simulink model "TV_Sim_Track_Copia"  (R2025b)
settings: Solver=VariableStepAuto  StartTime=0.0  StopTime=20  RelTol=1e-3
values from neighbouring files (symbols this model uses):
  Ki_array = zeros(size(Vx_array))    [PID_analysis.m]    (also in PID_tuning.m)
  psi_ref = theta + pi/2    [init_skidpad.m]
  s_ref = linspace(0, circonferenza, 200)    [init_skidpad.m]
  Vx_array = 1:1:30    [PID_analysis.m]    (also in PID_tuning.m)
  x_ref = R * cos(theta)    [init_skidpad.m]
  y_ref = R * sin(theta)    [init_skidpad.m]
undefined symbols (not defined in the file or in its folder): vp
libraries: slpidlib x3
(part 1 of 2)
settings Model: Creator=roly2  LastModifiedBy=HP

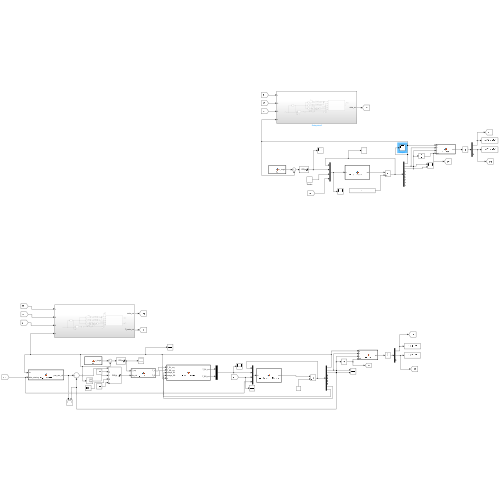
[thumbnail: Simulink's stored preview of the top-level diagram]
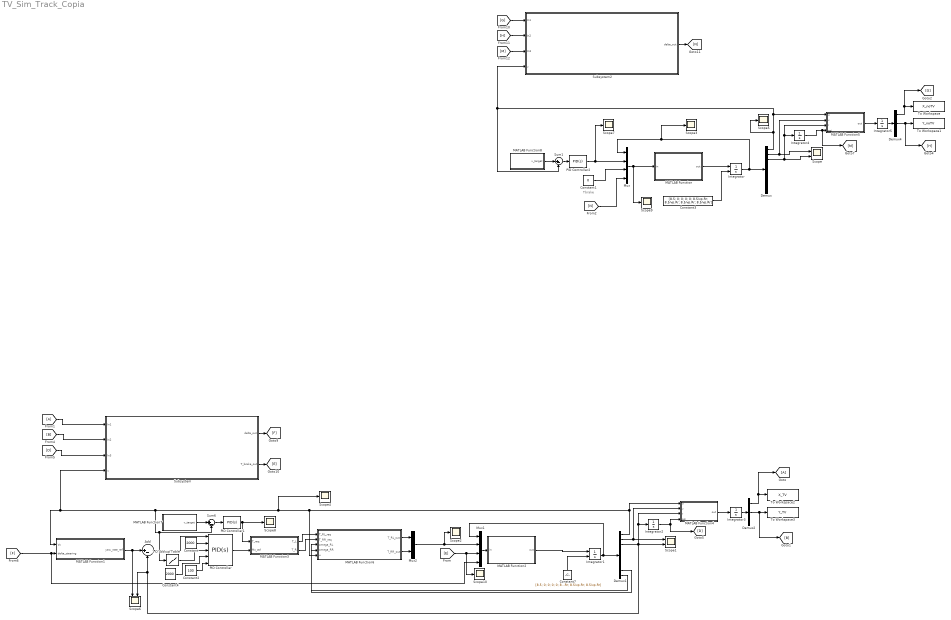
== system TV_Sim_Track_Copia ==
  note: Tbrake
  1-D Lookup Table : Lookup_n-D  NumberOfTableDimensions=1  BreakpointsForDimension1=Vx_array  Table=Ki_array  InternalRulePriority=Speed  RndMeth=Simplest
  Add : Sum  Inputs=|+-
  Constant : Constant  Value=2000
  Constant1 : Constant  Value=0
  Constant2 : Constant  Value=100
  Constant3 : Constant  Value=[8.5; 0; 0; 0; 0; 8.5/vp.Rr; 8.5/vp.Rr; 8.5/vp.Rr; 8.5/vp.Rr]
  Constant4 : Constant  Value=2000
  Constant7 : Constant  Value=[8.5; 0; 0; 0; 0; 8.5/vp.Rr; 8.5/vp.Rr; 8.5/vp.Rr; 8.5/vp.Rr]
  Demux : Demux  Outputs=9
  Demux1 : Demux  Outputs=9
  Demux2 : Demux  Outputs=3
  Demux4 : Demux  Outputs=3
  From1 : From
  Goto : Goto
  Integrator : Integrator  InitialConditionSource=external
  Integrator1 : Integrator  InitialConditionSource=external
  Integrator{2..5} (4 alike) : Integrator
  MATLAB Function : MATLAB Function  TreatAsAtomicUnit=on
  MATLAB Function1 : MATLAB Function  TreatAsAtomicUnit=on
  MATLAB Function2 : MATLAB Function  TreatAsAtomicUnit=on
  MATLAB Function3 : MATLAB Function  TreatAsAtomicUnit=on
  MATLAB Function4 : MATLAB Function  TreatAsAtomicUnit=on
  MATLAB Function5 : MATLAB Function  TreatAsAtomicUnit=on
  MATLAB Function6 : MATLAB Function  TreatAsAtomicUnit=on
  MATLAB Function7 : MATLAB Function  TreatAsAtomicUnit=on
  MATLAB Function8 : MATLAB Function  TreatAsAtomicUnit=on
  Mux : Mux
  Mux1 : Mux
  Mux2 : Mux  Inputs=2
  PID Controller : slpidlib/PID Controller  Controller=PID  Form=Parallel  TimeDomain=Continuous-time  UseExternalTs=off  SampleTime=-1  IntegratorMethod=Forward Euler  FilterMethod=Forward Euler  ControllerParametersSource=external  P=1500  I=12000  UseKiTs=off  D=0  UseExternalDerivativeSource=off  N=100  UseFilter=on  TunerSelectOption=Transfer Function Based (PID Tuner App)  ZeroCross=off  InitialConditionSource=internal  InitialConditionForIntegrator=0  InitialConditionForFilter=0  DifferentiatorICPrevScaledInput=0  ExternalReset=none  TrackingMode=off  Kt=1  LimitOutput=on  SatLimitsSource=internal  UpperSaturationLimit=1000  LowerSaturationLimit=-1000  LinearizeAsGain=on  AntiWindupMode=clamping  Kb=1  LimitIntegrator=off  UpperIntegratorSaturationLimit=inf  LowerIntegratorSaturationLimit=-inf  POutMin=[]  POutMax=[]  IOutMin=[]  IOutMax=[]  DOutMin=[]  DOutMax=[]  NOutMin=[]  NOutMax=[]  SumOutMin=[]  SumOutMax=[]  SaturationOutMin=[]  SaturationOutMax=[]  PParamMin=[]  PParamMax=[]  IParamMin=[]  IParamMax=[]  DParamMin=[]  DParamMax=[]  NParamMin=[]  NParamMax=[]  KbParamMin=[]  KbParamMax=[]  KtParamMin=[]  KtParamMax=[]  KbOutMin=[]  KbOutMax=[]  KtOutMin=[]  KtOutMax=[]  IntegratorOutMin=[]  IntegratorOutMax=[]  FilterOutMin=[]  FilterOutMax=[]  SumI1OutMin=[]  SumI1OutMax=[]  SumI2OutMin=[]  SumI2OutMax=[]  SumI3OutMin=[]  SumI3OutMax=[]  SumI4OutMin=[]  SumI4OutMax=[]  SumDOutMin=[]  SumDOutMax=[]  DifferentiatorOutMin=[]  DifferentiatorOutMax=[]  FilterDiffOutCoefMin=[]  FilterDiffOutCoefMax=[]  ReciprocalOutMin=[]  ReciprocalOutMax=[]  SumDenOutMin=[]  SumDenOutMax=[]  SumNumOutMin=[]  SumNumOutMax=[]  DivideOutMin=[]  DivideOutMax=[]  UdiffTsProdOutMin=[]  UdiffTsProdOutMax=[]  NTsProdOutMin=[]  NTsProdOutMax=[]  UintegralTsProdOutMin=[]  UintegralTsProdOutMax=[]  UngainTsProdOutMin=[]  UngainTsProdOutMax=[]  ClampingZeroOutDataTypeStr=Inherit: Inherit via back propagation  ClampingZeroOutMin=[]  ClampingZeroOutMax=[]  FilterDenConstantOutDataTypeStr=Inherit: Inherit via back propagation  FilterDenConstantOutMin=[]  FilterDenConstantOutMax=[]  PCopyOutDataTypeStr=Inherit: Inherit via back propagation  PCopyOutMin=[]  PCopyOutMax=[]  NCopyOutDataTypeStr=Inherit: Inherit via back propagation  NCopyOutMin=[]  NCopyOutMax=[]  IntegratorContinuousStateAttributes=''  IntegratorStateMustResolveToSignalObject=off  IntegratorRTWStateStorageClass=Auto  FilterContinuousStateAttributes=''  FilterStateMustResolveToSignalObject=off  FilterRTWStateStorageClass=Auto  ParallelPVariant=ExternalParameters  IdealPVariant=Disabled  IVariant=ExternalParameters  DVariant=ExternalParameters  IntegratorVariant=Continuous  SatVariant=Enabled  AWVariant=ContClampingParallel  PCopyVariant=Disabled  TRVariant=Disabled  FdbkBlocksVariant=Forward  IdealPFdbkVariant=Disabled  SatFdbkVariant=Disabled  DerivativeFilterVariant=ContFilter  NVariant=ExternalParameters  NCopyVariant=Disabled  FilterICVariant=InternalICsFilter  IntegratorICVariant=InternalICs  ExternalResetVariant=Disabled  TRSumVariant=Passthrough  SumFdbkVariant=Disabled  SumVariant=Sum_PID  TsampFilterVariant=InternalTs  TsampNgainVariant=Passthrough  TsampIntegralVariant=Disabled_SignalSpec  ExternalSaturationOutDataTypeStr=Inherit: Same as second input  DerivativeSourceVariant=ErrorSignal  PreIntVariant=InternalPreInt
  PID Controller1 : slpidlib/PID Controller  Controller=PID  Form=Parallel  TimeDomain=Continuous-time  UseExternalTs=off  SampleTime=-1  IntegratorMethod=Forward Euler  FilterMethod=Forward Euler  ControllerParametersSource=internal  P=2000  I=3  UseKiTs=off  D=0  UseExternalDerivativeSource=off  N=100  UseFilter=on  TunerSelectOption=Transfer Function Based (PID Tuner App)  InitialConditionSource=internal  InitialConditionForIntegrator=0  InitialConditionForFilter=0  DifferentiatorICPrevScaledInput=0  ExternalReset=none  TrackingMode=off  Kt=1  LimitOutput=on  SatLimitsSource=internal  UpperSaturationLimit=800  LowerSaturationLimit=-8000  LinearizeAsGain=on  AntiWindupMode=clamping  Kb=1  LimitIntegrator=off  UpperIntegratorSaturationLimit=inf  LowerIntegratorSaturationLimit=-inf  POutMin=[]  POutMax=[]  IOutMin=[]  IOutMax=[]  DOutMin=[]  DOutMax=[]  NOutMin=[]  NOutMax=[]  SumOutMin=[]  SumOutMax=[]  SaturationOutMin=[]  SaturationOutMax=[]  PParamMin=[]  PParamMax=[]  IParamMin=[]  IParamMax=[]  DParamMin=[]  DParamMax=[]  NParamMin=[]  NParamMax=[]  KbParamMin=[]  KbParamMax=[]  KtParamMin=[]  KtParamMax=[]  KbOutMin=[]  KbOutMax=[]  KtOutMin=[]  KtOutMax=[]  IntegratorOutMin=[]  IntegratorOutMax=[]  FilterOutMin=[]  FilterOutMax=[]  SumI1OutMin=[]  SumI1OutMax=[]  SumI2OutMin=[]  SumI2OutMax=[]  SumI3OutMin=[]  SumI3OutMax=[]  SumI4OutMin=[]  SumI4OutMax=[]  SumDOutMin=[]  SumDOutMax=[]  DifferentiatorOutMin=[]  DifferentiatorOutMax=[]  FilterDiffOutCoefMin=[]  FilterDiffOutCoefMax=[]  ReciprocalOutMin=[]  ReciprocalOutMax=[]  SumDenOutMin=[]  SumDenOutMax=[]  SumNumOutMin=[]  SumNumOutMax=[]  DivideOutMin=[]  DivideOutMax=[]  UdiffTsProdOutMin=[]  UdiffTsProdOutMax=[]  NTsProdOutMin=[]  NTsProdOutMax=[]  UintegralTsProdOutMin=[]  UintegralTsProdOutMax=[]  UngainTsProdOutMin=[]  UngainTsProdOutMax=[]  ClampingZeroOutDataTypeStr=Inherit: Inherit via back propagation  ClampingZeroOutMin=[]  ClampingZeroOutMax=[]  FilterDenConstantOutDataTypeStr=Inherit: Inherit via back propagation  FilterDenConstantOutMin=[]  FilterDenConstantOutMax=[]  PCopyOutDataTypeStr=Inherit: Inherit via back propagation  PCopyOutMin=[]  PCopyOutMax=[]  NCopyOutDataTypeStr=Inherit: Inherit via back propagation  NCopyOutMin=[]  NCopyOutMax=[]  IntegratorContinuousStateAttributes=''  IntegratorStateMustResolveToSignalObject=off  IntegratorRTWStateStorageClass=Auto  FilterContinuousStateAttributes=''  FilterStateMustResolveToSignalObject=off  FilterRTWStateStorageClass=Auto  ParallelPVariant=InternalParameters  IdealPVariant=Disabled  IVariant=InternalParameters  DVariant=InternalParameters  IntegratorVariant=Continuous  SatVariant=Enabled  AWVariant=ContClampingParallel  PCopyVariant=Disabled  TRVariant=Disabled  FdbkBlocksVariant=Forward  IdealPFdbkVariant=Disabled  SatFdbkVariant=Disabled  DerivativeFilterVariant=ContFilter  NVariant=InternalParameters  NCopyVariant=Disabled  FilterICVariant=InternalICsFilter  IntegratorICVariant=InternalICs  ExternalResetVariant=Disabled  TRSumVariant=Passthrough  SumFdbkVariant=Disabled  SumVariant=Sum_PID  TsampFilterVariant=InternalTs  TsampNgainVariant=Passthrough  TsampIntegralVariant=Disabled_SignalSpec  ExternalSaturationOutDataTypeStr=Inherit: Same as second input  DerivativeSourceVariant=ErrorSignal  PreIntVariant=InternalPreInt
  PID Controller2 : slpidlib/PID Controller  Controller=PID  Form=Parallel  TimeDomain=Continuous-time  UseExternalTs=off  SampleTime=-1  IntegratorMethod=Forward Euler  FilterMethod=Forward Euler  ControllerParametersSource=internal  P=50  I=3  UseKiTs=off  D=0  UseExternalDerivativeSource=off  N=100  UseFilter=on  TunerSelectOption=Transfer Function Based (PID Tuner App)  InitialConditionSource=internal  InitialConditionForIntegrator=0  InitialConditionForFilter=0  DifferentiatorICPrevScaledInput=0  ExternalReset=none  TrackingMode=off  Kt=1  LimitOutput=on  SatLimitsSource=internal  UpperSaturationLimit=800  LowerSaturationLimit=-8000  LinearizeAsGain=on  AntiWindupMode=clamping  Kb=1  LimitIntegrator=off  UpperIntegratorSaturationLimit=inf  LowerIntegratorSaturationLimit=-inf  POutMin=[]  POutMax=[]  IOutMin=[]  IOutMax=[]  DOutMin=[]  DOutMax=[]  NOutMin=[]  NOutMax=[]  SumOutMin=[]  SumOutMax=[]  SaturationOutMin=[]  SaturationOutMax=[]  PParamMin=[]  PParamMax=[]  IParamMin=[]  IParamMax=[]  DParamMin=[]  DParamMax=[]  NParamMin=[]  NParamMax=[]  KbParamMin=[]  KbParamMax=[]  KtParamMin=[]  KtParamMax=[]  KbOutMin=[]  KbOutMax=[]  KtOutMin=[]  KtOutMax=[]  IntegratorOutMin=[]  IntegratorOutMax=[]  FilterOutMin=[]  FilterOutMax=[]  SumI1OutMin=[]  SumI1OutMax=[]  SumI2OutMin=[]  SumI2OutMax=[]  SumI3OutMin=[]  SumI3OutMax=[]  SumI4OutMin=[]  SumI4OutMax=[]  SumDOutMin=[]  SumDOutMax=[]  DifferentiatorOutMin=[]  DifferentiatorOutMax=[]  FilterDiffOutCoefMin=[]  FilterDiffOutCoefMax=[]  ReciprocalOutMin=[]  ReciprocalOutMax=[]  SumDenOutMin=[]  SumDenOutMax=[]  SumNumOutMin=[]  SumNumOutMax=[]  DivideOutMin=[]  DivideOutMax=[]  UdiffTsProdOutMin=[]  UdiffTsProdOutMax=[]  NTsProdOutMin=[]  NTsProdOutMax=[]  UintegralTsProdOutMin=[]  UintegralTsProdOutMax=[]  UngainTsProdOutMin=[]  UngainTsProdOutMax=[]  ClampingZeroOutDataTypeStr=Inherit: Inherit via back propagation  ClampingZeroOutMin=[]  ClampingZeroOutMax=[]  FilterDenConstantOutDataTypeStr=Inherit: Inherit via back propagation  FilterDenConstantOutMin=[]  FilterDenConstantOutMax=[]  PCopyOutDataTypeStr=Inherit: Inherit via back propagation  PCopyOutMin=[]  PCopyOutMax=[]  NCopyOutDataTypeStr=Inherit: Inherit via back propagation  NCopyOutMin=[]  NCopyOutMax=[]  IntegratorContinuousStateAttributes=''  IntegratorStateMustResolveToSignalObject=off  IntegratorRTWStateStorageClass=Auto  FilterContinuousStateAttributes=''  FilterStateMustResolveToSignalObject=off  FilterRTWStateStorageClass=Auto  ParallelPVariant=InternalParameters  IdealPVariant=Disabled  IVariant=InternalParameters  DVariant=InternalParameters  IntegratorVariant=Continuous  SatVariant=Enabled  AWVariant=ContClampingParallel  PCopyVariant=Disabled  TRVariant=Disabled  FdbkBlocksVariant=Forward  IdealPFdbkVariant=Disabled  SatFdbkVariant=Disabled  DerivativeFilterVariant=ContFilter  NVariant=InternalParameters  NCopyVariant=Disabled  FilterICVariant=InternalICsFilter  IntegratorICVariant=InternalICs  ExternalResetVariant=Disabled  TRSumVariant=Passthrough  SumFdbkVariant=Disabled  SumVariant=Sum_PID  TsampFilterVariant=InternalTs  TsampNgainVariant=Passthrough  TsampIntegralVariant=Disabled_SignalSpec  ExternalSaturationOutDataTypeStr=Inherit: Same as second input  DerivativeSourceVariant=ErrorSignal  PreIntVariant=InternalPreInt
  Scope : Scope  NumInputPorts=2
      settings: ActiveDisplayYMinimum=-0.036171963019396312  ActiveDisplayYMaximum=0.32541321822804137
  Scope1 : Scope  NumInputPorts=2
      settings: ActiveDisplayYMinimum=-0.20199456045323017  ActiveDisplayYMaximum=0.60254469008079159
  Scope{2..5,7..10} (8 alike) : Scope
      Scope10 settings: ActiveDisplayYMinimum=-1  ActiveDisplayYMaximum=1  DataLoggingVariableName=ScopeData10
      Scope2 settings: ActiveDisplayYMinimum=-54.565881529047566  ActiveDisplayYMaximum=241.09293376142816  DataLoggingVariableName=ScopeData2
      Scope3 settings: ActiveDisplayYMinimum=-12.645443098724071  ActiveDisplayYMaximum=111.73678774278743  DataLoggingVariableName=ScopeData3
      Scope4 settings: ActiveDisplayYMinimum=-115.18294853972765  ActiveDisplayYMaximum=23.840986492179059  DataLoggingVariableName=ScopeData4
      Scope5 settings: ActiveDisplayYMinimum=7.8538069739436995  ActiveDisplayYMaximum=8.5717992251173669  DataLoggingVariableName=ScopeData5
      Scope7 settings: ActiveDisplayYMinimum=-3.3845352985098125  ActiveDisplayYMaximum=43.431126970490176  DataLoggingVariableName=ScopeData7
      Scope8 settings: ActiveDisplayYMinimum=-132.10801998182529  ActiveDisplayYMaximum=486.27732365321947  DataLoggingVariableName=ScopeData8
      Scope9 settings: ActiveDisplayYMinimum=-8.521232283481865  ActiveDisplayYMaximum=11.017708574192625  DataLoggingVariableName=ScopeData9
  Scope6 : Scope  NumInputPorts=2
      settings: ActiveDisplayYMinimum=-0.14426470588235293  ActiveDisplayYMaximum=1.2983823529411767  DataLoggingVariableName=ScopeData6
  Subsystem : Subsystem
  Subsystem2 : Subsystem
  Sum1 : Sum  Inputs=|+-
  Sum6 : Sum  Inputs=|+-
  To Workspace : ToWorkspace  VariableName=X_noTV  SaveFormat=Timeseries  SampleTime=-1
      settings: Save2DSignal=2-D array (concatenate along first dimension)
  To Workspace1 : ToWorkspace  VariableName=Y_noTV  SaveFormat=Timeseries  SampleTime=-1
      settings: Save2DSignal=2-D array (concatenate along first dimension)
  To Workspace2 : ToWorkspace  VariableName=X_TV  SaveFormat=Timeseries  SampleTime=-1
      settings: Save2DSignal=2-D array (concatenate along first dimension)
  To Workspace3 : ToWorkspace  VariableName=Y_TV  SaveFormat=Timeseries  SampleTime=-1
      settings: Save2DSignal=2-D array (concatenate along first dimension)
  wires:
  Add/1 -> PID Controller/1
  Constant7/1 -> Integrator1/2
  Demux2/1 -> Goto/1, To Workspace2/1
  MATLAB Function2/1(out) -> Integrator1/1
  Integrator3/1 -> Demux2/1
  Integrator1/1 -> Demux1/1, Mux1/1
  Demux2/2 -> [B], To Workspace3/1
  Integrator2/1 -> [D], MATLAB Function4/4(psi)
  Demux1/2 -> MATLAB Function4/2(v), Scope1/1
  MATLAB Function4/1(out) -> Integrator3/1
  Mux1/1 -> MATLAB Function2/1(in)
  Demux1/3 -> Add/2, Scope6/2, Integrator2/1, MATLAB Function4/3(r), Scope1/2
  Integrator4/1 -> [M], MATLAB Function5/4(psi)
  Integrator5/1 -> Demux4/1
  Integrator/1 -> Demux/1, Scope3/1, Mux/1
  Constant1/1 -> Mux/3
  MATLAB Function5/1(out) -> Integrator5/1
  Demux4/2 -> [H], To Workspace1/1
  Mux/1 -> Scope9/1, MATLAB Function/1(in)
  Constant3/1 -> Integrator/2
  MATLAB Function/1(out) -> Integrator/1
  Demux/3 -> Integrator4/1, MATLAB Function5/3(r), Scope/2
  Demux4/1 -> [G], To Workspace/1
  Demux/2 -> MATLAB Function5/2(v), Scope/1
  PID Controller/1 -> MATLAB Function3/2(Mz_ctrl)
  Mux2/1 -> Mux1/2, Scope2/1
  MATLAB Function3/2(T_R) -> MATLAB Function6/2(T_RR_req)
  MATLAB Function3/1(T_L) -> MATLAB Function6/1(T_RL_req)
  Demux1/8 -> MATLAB Function6/3(omega_RL)
  Demux1/9 -> MATLAB Function6/4(omega_RR)
  MATLAB Function6/1(T_RL_out) -> Mux2/1
  MATLAB Function6/2(T_RR_out) -> Mux2/2
  MATLAB Function1/1(yaw_rate_ref) -> Add/1, Scope6/1
  [F] -> Mux1/4, MATLAB Function1/2(delta_steering)
  MATLAB Function7/1(v_target) -> Sum6/1
  Sum6/1 -> PID Controller1/1
  PID Controller1/1 -> Scope8/1, MATLAB Function3/1(T_req)
  [N] -> Mux/4
  PID Controller2/1 -> Mux/2, Scope7/1
  Sum1/1 -> PID Controller2/1
  MATLAB Function8/1(v_target) -> Sum1/1
  Constant/1 -> PID Controller/2
  1-D Lookup Table/1 -> PID Controller/3
  Constant2/1 -> PID Controller/5
  Demux1/1 -> MATLAB Function4/1(u), 1-D Lookup Table/1, Sum6/2, MATLAB Function1/1(Vx), Subsystem/4(v), Scope4/1, MATLAB Function6/5(u)
  From1/1 -> Subsystem/1(In1)
  [B] -> Subsystem/2(In2)
  [D] -> Subsystem/3(In3)
  Subsystem/1(delta_out) -> [F]
  Subsystem/2(T_brake_out) -> [E]
  [E] -> Scope10/1, Mux1/3
  [M] -> Subsystem2/3(In3)
  Demux/1 -> Scope5/1, Subsystem2/4(v), Sum1/2, MATLAB Function5/1(u)
  [H] -> Subsystem2/2(In2)
  Subsystem2/1(delta_out) -> [N]
  [G] -> Subsystem2/1(In1)
  Constant4/1 -> PID Controller/4

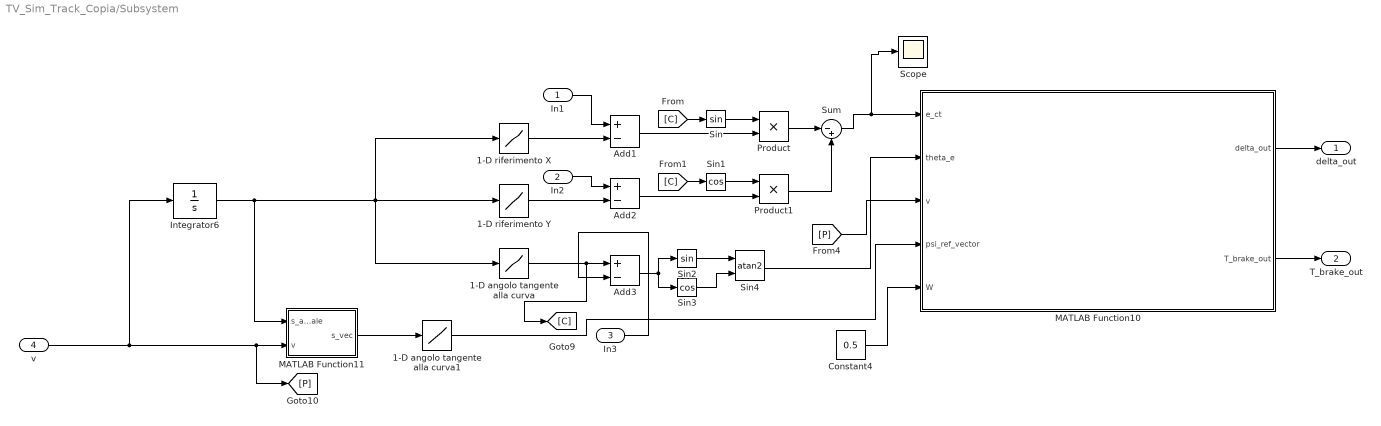
== system TV_Sim_Track_Copia/Subsystem ==
  In1 : Inport
  In2 : Inport  Port=2
  In3 : Inport  Port=3
  v : Inport  Port=4
  1-D angolo tangente alla curva : Lookup_n-D  NumberOfTableDimensions=1  BreakpointsForDimension1=s_ref  Table=psi_ref  ExtrapMethod=Clip  InternalRulePriority=Speed  RndMeth=Simplest
  1-D angolo tangente alla curva1 : Lookup_n-D  NumberOfTableDimensions=1  BreakpointsForDimension1=s_ref  Table=psi_ref  ExtrapMethod=Clip  InternalRulePriority=Speed  RndMeth=Simplest
  1-D riferimento X : Lookup_n-D  NumberOfTableDimensions=1  BreakpointsForDimension1=s_ref  Table=x_ref  ExtrapMethod=Clip  InternalRulePriority=Speed  RndMeth=Simplest
  1-D riferimento Y : Lookup_n-D  NumberOfTableDimensions=1  BreakpointsForDimension1=s_ref  Table=y_ref  ExtrapMethod=Clip  InternalRulePriority=Speed  RndMeth=Simplest
  Add1 : Sum  Inputs=+-
  Add2 : Sum  Inputs=+-
  Add3 : Sum  Inputs=+-
  Constant4 : Constant  Value=0.5
  Integrator6 : Integrator  UpperSaturationLimit=94.2478  LowerSaturationLimit=0
  MATLAB Function10 : MATLAB Function  TreatAsAtomicUnit=on
  MATLAB Function11 : MATLAB Function  TreatAsAtomicUnit=on
  Product : Product
  Product1 : Product
  Scope : Scope
      settings: ActiveDisplayYMinimum=-1  ActiveDisplayYMaximum=1  DataLoggingVariableName=ScopeData11
  Sin : Trigonometry
  Sin1 : Trigonometry  Operator=cos
  Sin2 : Trigonometry
  Sin3 : Trigonometry  Operator=cos
  Sin4 : Trigonometry  Operator=atan2
  Sum : Sum  Inputs=|-+
  delta_out : Outport
  T_brake_out : Outport  Port=2
  wires:
  v/1 -> Integrator6/1, [P], MATLAB Function11/2(v)
  Sin3/1 -> Sin4/2
  In1/1 -> Add1/1
  Sin4/1 -> MATLAB Function10/2(theta_e)
  MATLAB Function10/2(T_brake_out) -> T_brake_out/1
  1-D angolo tangente alla curva/1 -> [C], Add3/1
  [P] -> MATLAB Function10/3(v)
  1-D riferimento Y/1 -> Add2/2
  Sin2/1 -> Sin4/1
  Product/1 -> Sum/1
  [C] -> Sin1/1
  Add2/1 -> Product1/2
  Product1/1 -> Sum/2
  In2/1 -> Add2/1
  1-D angolo tangente alla curva1/1 -> MATLAB Function10/4(psi_ref_vector)
  Sin/1 -> Product/1
  Add3/1 -> Sin3/1, Sin2/1
  Add1/1 -> Product/2
  Sin1/1 -> Product1/1
  MATLAB Function11/1(s_vec) -> 1-D angolo tangente alla curva1/1
  1-D riferimento X/1 -> Add1/2
  In3/1 -> Add3/2
  Sum/1 -> Scope/1, MATLAB Function10/1(e_ct)
  [C] -> Sin/1
  Constant4/1 -> MATLAB Function10/5(W)
  MATLAB Function10/1(delta_out) -> delta_out/1
  Integrator6/1 -> MATLAB Function11/1(s_attuale), 1-D angolo tangente alla curva/1, 1-D riferimento X/1, 1-D riferimento Y/1

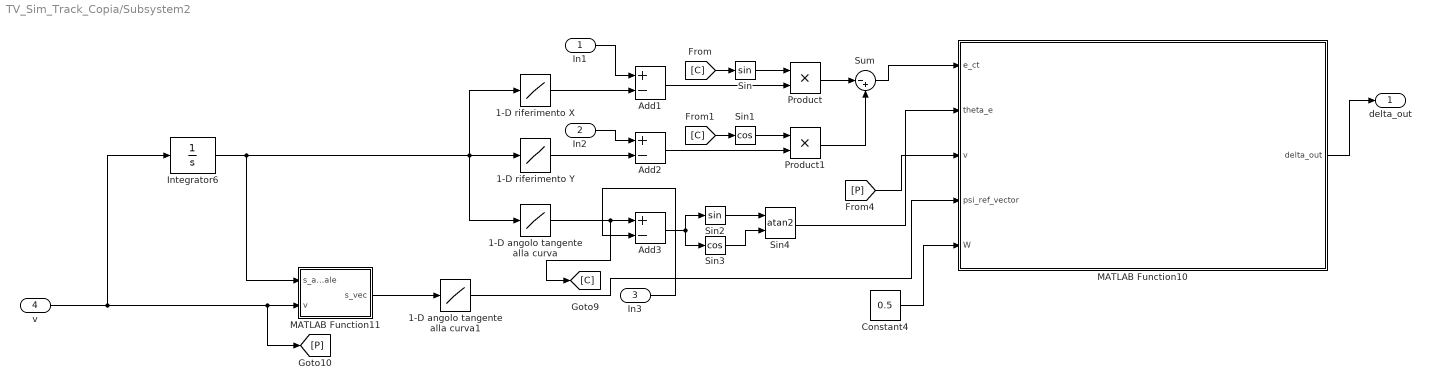
== system TV_Sim_Track_Copia/Subsystem2 ==
  In1 : Inport
  In2 : Inport  Port=2
  In3 : Inport  Port=3
  v : Inport  Port=4
  1-D angolo tangente alla curva : Lookup_n-D  NumberOfTableDimensions=1  BreakpointsForDimension1=s_ref  Table=psi_ref  ExtrapMethod=Clip  InternalRulePriority=Speed  RndMeth=Simplest
  1-D angolo tangente alla curva1 : Lookup_n-D  NumberOfTableDimensions=1  BreakpointsForDimension1=s_ref  Table=psi_ref  ExtrapMethod=Clip  InternalRulePriority=Speed  RndMeth=Simplest
  1-D riferimento X : Lookup_n-D  NumberOfTableDimensions=1  BreakpointsForDimension1=s_ref  Table=x_ref  ExtrapMethod=Clip  InternalRulePriority=Speed  RndMeth=Simplest
  1-D riferimento Y : Lookup_n-D  NumberOfTableDimensions=1  BreakpointsForDimension1=s_ref  Table=y_ref  ExtrapMethod=Clip  InternalRulePriority=Speed  RndMeth=Simplest
  Add1 : Sum  Inputs=+-
  Add2 : Sum  Inputs=+-
  Add3 : Sum  Inputs=+-
  Constant4 : Constant  Value=0.5
  Integrator6 : Integrator  UpperSaturationLimit=94.2478  LowerSaturationLimit=0
  MATLAB Function10 : MATLAB Function  TreatAsAtomicUnit=on
  MATLAB Function11 : MATLAB Function  TreatAsAtomicUnit=on
  Product : Product
  Product1 : Product
  Sin : Trigonometry
  Sin1 : Trigonometry  Operator=cos
  Sin2 : Trigonometry
  Sin3 : Trigonometry  Operator=cos
  Sin4 : Trigonometry  Operator=atan2
  Sum : Sum  Inputs=|-+
  delta_out : Outport
  wires:
  v/1 -> Integrator6/1, [P], MATLAB Function11/2(v)
  Sin3/1 -> Sin4/2
  In1/1 -> Add1/1
  Sin4/1 -> MATLAB Function10/2(theta_e)
  1-D angolo tangente alla curva/1 -> [C], Add3/1
  [P] -> MATLAB Function10/3(v)
  1-D riferimento Y/1 -> Add2/2
  Integrator6/1 -> 1-D angolo tangente alla curva/1, 1-D riferimento X/1, 1-D riferimento Y/1, MATLAB Function11/1(s_attuale)
  Sin2/1 -> Sin4/1
  Product/1 -> Sum/1
  [C] -> Sin1/1
  Add2/1 -> Product1/2
  Product1/1 -> Sum/2
  In2/1 -> Add2/1
  1-D angolo tangente alla curva1/1 -> MATLAB Function10/4(psi_ref_vector)
  Sin/1 -> Product/1
  Add3/1 -> Sin3/1, Sin2/1
  Add1/1 -> Product/2
  Sin1/1 -> Product1/1
  MATLAB Function11/1(s_vec) -> 1-D angolo tangente alla curva1/1
  1-D riferimento X/1 -> Add1/2
  In3/1 -> Add3/2
  Sum/1 -> MATLAB Function10/1(e_ct)
  [C] -> Sin/1
  Constant4/1 -> MATLAB Function10/5(W)
  MATLAB Function10/1(delta_out) -> delta_out/1

== matlab function TV_Sim_Track_Copia/Subsystem/MATLAB Function10 ==
  data: e_ct input; delta_out output; T_brake_out output; theta_e input; v input; psi_ref_vector input; W input
function [delta_out, T_brake_out] = fcn(e_ct, theta_e, v, psi_ref_vector, W)
    % --- PARAMETRI DI CONFIGURAZIONE ---
    N = length(psi_ref_vector); % Numero di punti futuri (es. 10)
    dt = 0.1;                   % Passo temporale della previsione [s]
    
    % Margine di sicurezza: l'auto cercherà di stare entro questo limite
    % Se W=10m, Lat_Limit sarà 4.7m (lasciando 30cm dal bordo)
    Lat_Limit = (W/2) - 0.3; 

    % --- 1. PREVISIONE DEL FUTURO (ORIZZONTE N) ---
    % Inizializziamo le variabili per la simulazione interna
    future_e_ct = zeros(1, N);
    temp_e = e_ct;
    temp_theta = theta_e;
    
for k = 1:N
    % Calcola la differenza angolare
    diff_angle = temp_theta - psi_ref_vector(k);
    
    % CORREZIONE WRAP-AROUND: mantiene l'angolo tra -pi e pi
    diff_angle = atan2(sin(diff_angle), cos(diff_angle));
    
    % Usa l'angolo corretto per la previsione
    temp_e = temp_e + v * sin(diff_angle) * dt;
    future_e_ct(k) = temp_e;
end

    % --- 2. LOGICA DI CONTROLLO STERZO (FEEDBACK) ---
    % Usiamo una base simile allo Stanley per l'inseguimento normale
    k_stanley = 0.5;
    k_soft = 1.0;
    delta_feedback = theta_e - atan2(k_stanley * e_ct, v + k_soft);

    % --- 3. LOGICA DI VINCOLO (THE "HARD" CONSTRAINT) ---
    % Troviamo l'errore massimo previsto nell'orizzonte
    max_predicted_error = max(abs(future_e_ct));
    
    if max_predicted_error > Lat_Limit
        % --- SE L'AUTO PREVEDE DI USCIRE ---
        
        % A. Calcoliamo quanto stiamo violando il limite
        violazione = max_predicted_error - Lat_Limit;
        
        % B. FRENO OBBLIGATORIO: Più la violazione è grande, più frena.
        % Questo riduce v e "stringe" la traiettoria fisicamente.
        T_brake_out = 0; %2500 * violazione; 
        
        % C. STERZO DI EMERGENZA: Aumentiamo il guadagno per chiudere la curva
        delta_out = delta_feedback * (1 + 2 * violazione);
    else
        % --- TRAIETTORIA SICURA ---
        T_brake_out = 0;
        delta_out = delta_feedback;
    end

    % --- 4. SATURAZIONI FISICHE ---
    % Limite sterzo (es. 35 gradi)
    delta_out = max(min(delta_out, 0.6), -0.6);
    
    % Limite frenata massima (Nm)
    T_brake_out = max(min(T_brake_out, 4000), 0);
end

== matlab function TV_Sim_Track_Copia/Subsystem/MATLAB Function11 ==
  data: s_attuale input; s_vec output; v input
function s_vec = fcn(s_attuale, v)
    dt = 0.1; % Passo temporale (prevediamo i prossimi 10 decimi di secondo)
    % Creiamo un vettore: [s, s+v*0.1, s+v*0.2, ..., s+v*0.9]
    s_vec = s_attuale + v * dt * (0:9); 
end

== matlab function TV_Sim_Track_Copia/Subsystem2/MATLAB Function11 ==
  data: s_attuale input; s_vec output; v input
function s_vec = fcn(s_attuale, v)
    dt = 0.1; % Passo temporale (prevediamo i prossimi 10 decimi di secondo)
    % Creiamo un vettore: [s, s+v*0.1, s+v*0.2, ..., s+v*0.9]
    s_vec = s_attuale + v * dt * (0:9); 
end

== matlab function TV_Sim_Track_Copia/MATLAB Function1 ==
  data: Vx input; delta_steering input; yaw_rate_ref output; vp parameter
function yaw_rate_ref = ref_generator(Vx, delta_steering, vp)

% --- 1. PARAMETRI E CONVERSIONI ---
% Stima del coefficiente d'attrito (es. 1.0 asciutto, 0.7 umido)
% In futuro questo valore potrà arrivare da uno stimatore
mu = 1.0;

K_tf_deg = 1150;
K_tr_deg = 1010;
K_tf = K_tf_deg * (180/pi); 
K_tr = K_tr_deg * (180/pi); 

K_us = (vp.m / vp.l)*(vp.a2/K_tf - vp.a1/K_tr);

delta = delta_steering * vp.tau1;

% --- 2. RIFERIMENTO LINEARE (Desired Handling) ---
% Eq. (1) del paper: Comportamento ideale se avessimo grip infinito [cite: 2044]
% Protezione per Vx molto bassi per evitare divisioni per zero instabili
Vx_safe = max(abs(Vx), 1.0);

r_linear = Vx / (vp.l*(1 + K_us * Vx^2)) * delta;

% --- 3. SATURAZIONE FISICA (Safety/Grip Limit) ---
% Il paper spiega che il limite è dato dall'attrito disponibile 
% Massima accelerazione laterale sostenibile (in m/s^2)
ay_max = mu * vp.g;

% Massima velocità di imbardata possibile a questa velocità
% Dalla relazione: ay = V * r  -->  r_max = ay_max / V
r_max_phys = ay_max / Vx_safe;

% --- 4. OUTPUT FINALE (Logica Min/Max) ---
% Il riferimento è il minimo tra quello che "vorrebbe" il pilota (lineare)
% e quello che la fisica "permette" (limite saturato).

% Manteniamo il segno originale della richiesta
sign_r = sign(r_linear);

% Se la richiesta lineare supera il limite fisico, tagliamo al limite.
if abs(r_linear) > r_max_phys
    yaw_rate_ref = sign_r * r_max_phys;
else
    yaw_rate_ref = r_linear;
end

% (Opzionale Avanzato): Per mimare l'esponenziale del paper,
% si potrebbe usare una tanh() per una transizione più morbida vicino al limite,
% ma la saturazione secca (if/else) sopra è più sicura per iniziare.


end

== matlab function TV_Sim_Track_Copia/MATLAB Function ==
  data: in input size=12; out output; vp parameter
function out  = Vehicle_model_NL(in, vp)
% Modello del veicolo non lineare

u = in(1);
v = in(2);
r = in(3);
nu = in(4);
epsilon = in(5);
omega11 = in(6);
omega12 = in(7);
omega21 = in(8);
omega22 = in(9);
% Coppia motrice [Nm]
Tdrive = in(10);
% Coppia frenante [Nm]
Tbrake = in(11);
% Angolo di sterzo [rad]
deltav = in(12);


% ModelloVeicolo_2025/2026

% 2) Definizione dei limiti sugli stati

u_lim = 1/u*[0 vp.Vmax]; % Questo è abbastanza chiaro, in caso va solo cambiata la scalatura
v_lim = 1/v*[-10 10]; % Questo si cerca di tenerlo attorno a 1
r_lim = 1/r*[-10 10]; % Qui mettiamoci un pi/2 
nu_lim = 1/nu*[-0.875 0.875]; %Per skid
%nu_lim = 1/nu*[-1 1]; % Questo in teoria permette di specificare la largezza del circuito, assunta costante. Dovrebbe esserci il modo di mettere una distanza variabile ma è follia, messo a 1
epsilon_lim = 1/epsilon*[-pi/4 pi/4]; % Un po' strano ma in realtà è solo pi/4
% Le velocità angolari abbastanza semplici, fermo al minimo, Vmax/u al massimo
omega11_lim = 1/omega11*[0 vp.Vmax/vp.Rr];
omega12_lim = 1/omega12*[0 vp.Vmax/vp.Rr];
omega21_lim = 1/omega21*[0 vp.Vmax/vp.Rr];
omega22_lim = 1/omega22*[0 vp.Vmax/vp.Rr];

% 3) Raggruppamento

% Vettore degli stati 
X = [u; v; r; nu; epsilon; omega11; omega12; omega21; omega22];
% Limiti
X_lim = [u_lim;v_lim;r_lim;nu_lim;epsilon_lim;omega11_lim;omega12_lim;omega21_lim;omega22_lim];
X_min = X_lim(:,1);
X_max = X_lim(:,2);

% Differernziale similmeccanico aperto ***********
TdriveR = (Tdrive)/2; 
TdriveL = (Tdrive)/2;

% 2) Definizione dei limiti sui controlli + Frenata rigenerativa

TdriveR_lim = 1/TdriveR*[-vp.Tregenmax vp.Tdrivemax];
TdriveL_lim = 1/TdriveL*[-vp.Tregenmax vp.Tdrivemax];
Tbrake_lim = 1/Tbrake*[-vp.Tbrakemax 0];
deltav_lim = 1/deltav*[-pi/2 pi/2];

% 3) Raggruppamento

% Vettore dei controlli
U = [Tdrive; Tbrake; deltav];
% Limiti
U_lim = [TdriveR_lim;TdriveL_lim;Tbrake_lim;deltav_lim];
U_min = U_lim(:,1);
U_max = U_lim(:,2);

% Vincolo ulteriore sulla derivata dei controlli, sfrutta quello definito prima
%duk_ub = duk_ub./U;
%duk_lb = duk_lb./U;
%per ora sono come testo perchè non so quanto valgono queste derivate

% VARIABILI AUSILIARIE

% 1) Definizione simbolica deille variabili ausiliarie

% Trasferimento di carico longitudinale [N]
deltaZ = vp.m*vp.g*vp.h/vp.l;

% Trasferimento di carico laterale anteriore [N]
deltaZ1 = (((vp.kphi1/vp.kphi)*(vp.m*vp.g)*(vp.h-vp.qb)+(vp.m*vp.g*vp.a2/vp.l)*vp.q1+(vp.kphi1*vp.kphi2/vp.kphi)*((vp.m*vp.g*vp.a1/vp.l)*vp.q2/vp.kphi2p-(vp.m*vp.g*vp.a2/vp.l)*vp.q1/vp.kphi1p))*(1/vp.t1));

% Trasferimento di carico laterale posteriore [N]
deltaZ2 = (((vp.kphi1/vp.kphi)*(vp.m*vp.g)*(vp.h-vp.qb)+(vp.m*vp.g*vp.a1/vp.l)*vp.q1+(vp.kphi1*vp.kphi2/vp.kphi)*((vp.m*vp.g*vp.a2/vp.l)*vp.q2/vp.kphi2p-(vp.m*vp.g*vp.a1/vp.l)*vp.q1/vp.kphi1p))*(1/vp.t1));

% 2) Definizione dei limiti sulle variabili ausiliarie

deltaZ_lim = 1/deltaZ*[-2*vp.m*vp.g 2*vp.m*vp.g];
deltaZ1_lim = 1/deltaZ1*[-2*vp.m*vp.g 2*vp.m*vp.g];
deltaZ2_lim = 1/deltaZ2*[-2*vp.m*vp.g 2*vp.m*vp.g];

% 3) Raggruppamento

% Vettore delle variabili ausiliarie 
Zaus = [deltaZ;deltaZ1;deltaZ2];
% Limiti
Zaus_lim = [deltaZ_lim;deltaZ1_lim;deltaZ2_lim];
Zaus_min = Zaus_lim(:,1);
Zaus_max = Zaus_lim(:,2);

% EQUAZIONI 

% 1) Legge di sterzo

delta11 = -vp.delta10+vp.tau1*deltav+vp.eps1*(vp.t1/(2*vp.l))*(vp.t1*deltav)^2;
delta12 = vp.delta10+vp.tau1*deltav-vp.eps1*(vp.t1/(2*vp.l))*(vp.t1*deltav)^2;
delta21 = -vp.delta20+vp.tau2*deltav+vp.eps2*(vp.t2/(2*vp.l))*(vp.t2*deltav)^2;
delta22 = vp.delta20+vp.tau2*deltav-vp.eps2*(vp.t2/(2*vp.l))*(vp.t2*deltav)^2;

% 2) Velocità pneumatici sistema "Body

% FRONT LEFT
Vb11x = u-(r*vp.t1)/2; Vb11y = v+r*vp.a1;
% FRONT RIGHT
Vb12x = u+(r*vp.t1)/2; Vb12y = v+r*vp.a1;
% REAR LEFT
Vb21x = u-(r*vp.t2)/2; Vb21y = v-r*vp.a2;
% REAR RIGHT
Vb22x = u+(r*vp.t2)/2; Vb22y = v-r*vp.a2;

% 3) Angoli di assetto

% FRONT LEFT
beta11 = (v+r*vp.a1)/(u-r*vp.t1/2);
% FRONT RIGHT
beta12 = (v+r*vp.a1)/(u+r*vp.t1/2);
% REAR LEFT
beta21 = (v-r*vp.a2)/(u-r*vp.t2/2);
% REAR RIGHT
beta22 = (v-r*vp.a2)/(u+r*vp.t2/2);

% 3b) Velocità sistema "Wheel"

% FRONT LEFT
Vw11x = [cos(delta11) sin(delta11)]*[Vb11x;Vb11y];
Vw11y = [-sin(delta11) cos(delta11)]*[Vb11x;Vb11y];
% FRONT RIGHT
Vw12x = [cos(delta12) sin(delta12)]*[Vb12x;Vb12y];
Vw12y = [-sin(delta12) cos(delta12)]*[Vb12x;Vb12y];
% REAR LEFT
Vw21x = [cos(delta21) sin(delta21)]*[Vb21x;Vb21y];
Vw21y = [-sin(delta21) cos(delta21)]*[Vb21x;Vb21y];
% REAR RIGHT
Vw22x = [cos(delta22) sin(delta22)]*[Vb22x;Vb22y];
Vw22y = [-sin(delta22) cos(delta22)]*[Vb22x;Vb22y];

% 4) Angoli di deriva

% FRONT LEFT
alpha11 = delta11-beta11;
% FRONT RIGHT
alpha12 = delta12-beta12;
% REAR LEFT
alpha21 = delta21-beta21;
% REAR RIGHT
alpha22 = delta22-beta22;

% 5) Scorrimenti teorici

% Longitudinali
sigmax11 = (((u-r*vp.t1/2)*cos(delta11)+(v+r*vp.a1)*sin(delta11))-omega11*vp.Rr)/(omega11*vp.Rr);
sigmax12 = (((u+r*vp.t1/2)*cos(delta12)+(v+r*vp.a1)*sin(delta12))-omega12*vp.Rr)/(omega12*vp.Rr);
sigmax21 = (((u-r*vp.t2/2)*cos(delta21)+(v-r*vp.a2)*sin(delta21))-omega21*vp.Rr)/(omega21*vp.Rr);
sigmax22 = (((u+r*vp.t2/2)*cos(delta22)+(v-r*vp.a2)*sin(delta22))-omega22*vp.Rr)/(omega22*vp.Rr);
% Laterali
sigmay11 = ((v+r*vp.a1)*cos(delta11)-(u-r*vp.t1/2)*sin(delta11))/(omega11*vp.Rr);
sigmay12 = ((v+r*vp.a1)*cos(delta12)-(u+r*vp.t1/2)*sin(delta12))/(omega12*vp.Rr);
sigmay21 = ((v-r*vp.a2)*cos(delta21)-(u-r*vp.t2/2)*sin(delta21))/(omega21*vp.Rr);
sigmay22 = ((v-r*vp.a2)*cos(delta22)-(u+r*vp.t2/2)*sin(delta22))/(omega22*vp.Rr);

% 6) Scorrimenti pratici

% SR = slip ratio (quelli lungo x)
% SA = slip angle (quelli lungo y)
SR11 = -(sigmax11/(1+sigmax11));
SR12 = -(sigmax12/(1+sigmax12));
SR21 = -(sigmax21/(1+sigmax21));
SR22 = -(sigmax22/(1+sigmax22));
SA11 = -(sigmay11/(1+sigmax11));
SA12 = -(sigmay12/(1+sigmax12));
SA21 = -(sigmay21/(1+sigmax21));
SA22 = -(sigmay22/(1+sigmax22));

% 7) Aerodinamica

% Resistenza aerodinamica [N]
Xa = 0.5*vp.rho*vp.S*vp.Cx*u^2;

% Deportanza anteriore e posteriore [N]
Z1a = 0.5*vp.rho*vp.S*vp.Cz1*u^2;
Z2a = 0.5*vp.rho*vp.S*vp.Cz2*u^2;

% 8) Carichi sulle ruote

Z10 = vp.m*vp.g*vp.a2/vp.l;
Z20 = vp.m*vp.g*vp.a1/vp.l;

Fz11 = 0.5*(Z10+Z1a-deltaZ)-deltaZ1;
Fz12 = 0.5*(Z10+Z1a-deltaZ)+deltaZ1;
Fz21 = 0.5*(Z20+Z2a+deltaZ)-deltaZ2;
Fz22 = 0.5*(Z20+Z2a+deltaZ)+deltaZ2;

Dx11 = 2.05 * Fz11 - 1.9e-5 * Fz11^2;  % Picco Longitudinale
Dy11 = 1.86 * Fz11 - 2.6e-4 * Fz11^2;  % Picco Laterale
Dx12 = 2.05 * Fz12 - 1.9e-5 * Fz12^2;
Dy12 = 1.86 * Fz12 - 2.6e-4 * Fz12^2;
Dx21 = 2.05 * Fz21 - 1.9e-5 * Fz21^2;
Dy21 = 1.86 * Fz21 - 2.6e-4 * Fz21^2;
Dx22 = 2.05 * Fz22 - 1.9e-5 * Fz22^2;
Dy22 = 1.86 * Fz22 - 2.6e-4 * Fz22^2;

% --- 2. FORZE PURE (Magic Formula base) ---
% Fx0 (Longitudinale)
Bx=45.34; Cx=1.14; Ex=0.55;
Fx011 = Dx11 * sin(Cx * atan(Bx*SR11 - Ex*(Bx*SR11 - atan(Bx*SR11))));
Fx012 = Dx12 * sin(Cx * atan(Bx*SR12 - Ex*(Bx*SR12- atan(Bx*SR12))));
Fx021 = Dx21 * sin(Cx * atan(Bx*SR21 - Ex*(Bx*SR21 - atan(Bx*SR21))));
Fx022 = Dx22 * sin(Cx * atan(Bx*SR22 - Ex*(Bx*SR22 - atan(Bx*SR22))));
% Fy0 (Laterale)
By=20.74; Cy=1.20; Ey=0.48;
Fy011 = Dy11 * sin(Cy * atan(By*SA11 - Ey*(By*SA11 - atan(By*SA11))));
Fy012 = Dy12 * sin(Cy * atan(By*SA12 - Ey*(By*SA12 - atan(By*SA12))));
Fy021 = Dy21 * sin(Cy * atan(By*SA21 - Ey*(By*SA21 - atan(By*SA21))));
Fy022 = Dy22 * sin(Cy * atan(By*SA22 - Ey*(By*SA22 - atan(By*SA22))));
% --- 3. COMBINATO (Ovale di Attrito) ---
% Evita che il vettore forza superi il grip fisico disponibile
Rho = sqrt((Fx011/Dx11)^2 + (Fy011/Dy11)^2);
if Rho > 1
    Scale = 1/Rho;
    Fx11 = Fx011 * Scale;
    Fy11 = Fy011 * Scale;
else
    Fx11 = Fx011;
    Fy11 = Fy011;
end
Rho = sqrt((Fx012/Dx12)^2 + (Fy012/Dy12)^2);
if Rho > 1
    Scale = 1/Rho;
    Fx12 = Fx012 * Scale;
    Fy12 = Fy012 * Scale;
else
    Fx12 = Fx012;
    Fy12 = Fy012;
end
Rho = sqrt((Fx021/Dx21)^2 + (Fy021/Dy21)^2);
if Rho > 1
    Scale = 1/Rho;
    Fx21 = Fx021 * Scale;
    Fy21 = Fy021 * Scale;
else
    Fx21 = Fx021;
    Fy21 = Fy021;
end
Rho = sqrt((Fx022/Dx22)^2 + (Fy022/Dy22)^2);
if Rho > 1
    Scale = 1/Rho;
    Fx22 = Fx022 * Scale;
    Fy22 = Fy022 * Scale;
else
    Fx22 = Fx022;
    Fy22 = Fy022;
end
% --- 4. MOMENTI (Mz, Mx, My) ---
% Mz (Auto-allineamento) - Modellato con MF fittizia
Bmz=8.8; Cmz=2.4; Emz=0.95; Dmz11 = 0.023*Fz11 - 3e-6*Fz11^2;
Dmz12 = 0.023*Fz12 - 3e-6*Fz12^2;
Dmz21 = 0.023*Fz21 - 3e-6*Fz21^2;
Dmz22 = 0.023*Fz22 - 3e-6*Fz22^2;
Mz11_raw = -Dmz11 * sin(Cmz * atan(Bmz*SA11 - Emz*(Bmz*SA11 - atan(Bmz*SA11))));
Mz12_raw = -Dmz12 * sin(Cmz * atan(Bmz*SA12 - Emz*(Bmz*SA12 - atan(Bmz*SA12))));
Mz21_raw = -Dmz21 * sin(Cmz * atan(Bmz*SA21 - Emz*(Bmz*SA21 - atan(Bmz*SA21))));
Mz22_raw = -Dmz22 * sin(Cmz * atan(Bmz*SA22 - Emz*(Bmz*SA22 - atan(Bmz*SA22))));
Mz11 = Mz11_raw*(1-abs(SR11));
Mz12 = Mz12_raw*(1-abs(SR12));
Mz21 = Mz21_raw*(1-abs(SR21));
Mz22 = Mz22_raw*(1-abs(SR22));
% Mx (Ribaltante) - Lineare
Mx11 = -0.024 * Fy11;
Mx12 = -0.024 * Fy12;
Mx21 = -0.024 * Fy21;
Mx22 = -0.024 * Fy22;
% My (Rotolamento) - Costante
My11 = -sign(u) * (0.0024 * Fz11);
My12 = -sign(u) * (0.0024 * Fz12);
My21 = -sign(u) * (0.0024 * Fz21);
My22 = -sign(u) * (0.0024 * Fz22);

% Equazioni di supporto
X11 = Fx11*cos(delta11)-Fy11*sin(delta11);
X12 = Fx12*cos(delta12)-Fy12*sin(delta12);
X21 = Fx21*cos(delta21)-Fy21*sin(delta21);
X22 = Fx22*cos(delta22)-Fy22*sin(delta22);
Y11 = Fx11*sin(delta11)+Fy11*cos(delta11);
Y12 = Fx12*sin(delta12)+Fy12*cos(delta12);
Y21 = Fx21*sin(delta21)+Fy21*cos(delta21);
Y22 = Fx22*sin(delta22)+Fy22*cos(delta22);
X1 = (Fx11*cos(delta11)+Fx12*cos(delta12))-(Fy11*sin(delta11)+Fy12*sin(delta12));
X2 = (Fx21*cos(delta21)+Fx22*cos(delta22))-(Fy21*sin(delta21)+Fy22*sin(delta22));
Y1 = (Fy11*cos(delta11)+Fy12*cos(delta12))+(Fx11*sin(delta11)+Fx12*sin(delta12));
Y2 = (Fy21*cos(delta21)+Fy22*cos(delta22))+(Fx21*sin(delta21)+Fx22*sin(delta22));
deltaX1 = ((Fx12*cos(delta12)-Fx11*cos(delta11))-(Fy12*sin(delta12)-Fy11*sin(delta11)))/2;
deltaX2 = ((Fx22*cos(delta22)-Fx21*cos(delta21))-(Fy22*sin(delta22)-Fy21*sin(delta21)))/2;

% Ruote Anteriori (11 = FL, 12 = FR)
% Nelle Formula SAE a trazione posteriore, qui arriva solo la frenata
T11 = Tbrake / 4; 
T12 = Tbrake / 4;

% Ruote Posteriori (21 = RL, 22 = RR)
% Qui arriva la coppia motrice (Tdrive) divisa dal differenziale + la frenata
T21 = (Tdrive / 2) + (Tbrake / 4);
T22 = (Tdrive / 2) + (Tbrake / 4);

% Derivate
dot_u = (((X1+X2-Xa)/vp.m)+v*r);
dot_v = (((Y1+Y2)/vp.m)-u*r);
dot_r = ((Y1*vp.a1-Y2*vp.a2+deltaX1*vp.t1+deltaX2*vp.t2)/vp.Jz);
dot_nu = (u*sin(epsilon)+v*cos(epsilon));
dot_epsilon = r;
dot_omega11 = ((T11-Fx11*vp.Rr)/vp.tyre.IYY);
dot_omega12 = ((T12-Fx12*vp.Rr)/vp.tyre.IYY);
dot_omega21 = ((T21-Fx21*vp.Rr)/vp.tyre.IYY);
dot_omega22 = ((T22-Fx22*vp.Rr)/vp.tyre.IYY);
% Scalatura
dot_x = [dot_u; dot_v; dot_r; dot_nu; dot_epsilon; 
            dot_omega11; dot_omega12; dot_omega21; dot_omega22];

out = dot_x;

end

== matlab function TV_Sim_Track_Copia/MATLAB Function2 ==
  data: in input; out output; vp parameter
function out  = Vehicle_model_NL_cntrl(in, vp)
% Modello del veicolo non lineare

u = in(1);
v = in(2);
r = in(3);
nu = in(4);
epsilon = in(5);
omega11 = in(6);
omega12 = in(7);
omega21 = in(8);
omega22 = in(9);
% Coppie motrici [Nm]
TdriveL = in(10);
TdriveR = in(11);
% Coppia frenante [Nm]
Tbrake = in(12);
% Angolo di sterzo [rad]
deltav = in(13);


% ModelloVeicolo_2025/2026

% 2) Definizione dei limiti sugli stati

u_lim = 1/u*[0 vp.Vmax]; % Questo è abbastanza chiaro, in caso va solo cambiata la scalatura
v_lim = 1/v*[-10 10]; % Questo si cerca di tenerlo attorno a 1
r_lim = 1/r*[-10 10]; % Qui mettiamoci un pi/2 
nu_lim = 1/nu*[-0.875 0.875]; %Per skid
%nu_lim = 1/nu*[-1 1]; % Questo in teoria permette di specificare la largezza del circuito, assunta costante. Dovrebbe esserci il modo di mettere una distanza variabile ma è follia, messo a 1
epsilon_lim = 1/epsilon*[-pi/4 pi/4]; % Un po' strano ma in realtà è solo pi/4
% Le velocità angolari abbastanza semplici, fermo al minimo, Vmax/u al massimo
omega11_lim = 1/omega11*[0 vp.Vmax/vp.Rr];
omega12_lim = 1/omega12*[0 vp.Vmax/vp.Rr];
omega21_lim = 1/omega21*[0 vp.Vmax/vp.Rr];
omega22_lim = 1/omega22*[0 vp.Vmax/vp.Rr];

% 3) Raggruppamento

% Vettore degli stati 
X = [u; v; r; nu; epsilon; omega11; omega12; omega21; omega22];
% Limiti
X_lim = [u_lim;v_lim;r_lim;nu_lim;epsilon_lim;omega11_lim;omega12_lim;omega21_lim;omega22_lim];
X_min = X_lim(:,1);
X_max = X_lim(:,2);


% 2) Definizione dei limiti sui controlli + Frenata rigenerativa

TdriveR_lim = 1/TdriveR*[-vp.Tregenmax vp.Tdrivemax];
TdriveL_lim = 1/TdriveL*[-vp.Tregenmax vp.Tdrivemax];
Tbrake_lim = 1/Tbrake*[-vp.Tbrakemax 0];
deltav_lim = 1/deltav*[-pi/2 pi/2];

% 3) Raggruppamento

% Vettore dei controlli
U = [TdriveR; TdriveL; Tbrake; deltav];
% Limiti
U_lim = [TdriveR_lim;TdriveL_lim;Tbrake_lim;deltav_lim];
U_min = U_lim(:,1);
U_max = U_lim(:,2);

% Vincolo ulteriore sulla derivata dei controlli, sfrutta quello definito prima
%duk_ub = duk_ub./U;
%duk_lb = duk_lb./U;
%per ora sono come testo perchè non so quanto valgono queste derivate

% VARIABILI AUSILIARIE

% 1) Definizione simbolica deille variabili ausiliarie

% Trasferimento di carico longitudinale [N]
deltaZ = vp.m*vp.g*vp.h/vp.l;

% Trasferimento di carico laterale anteriore [N]
deltaZ1 = (((vp.kphi1/vp.kphi)*(vp.m*vp.g)*(vp.h-vp.qb)+(vp.m*vp.g*vp.a2/vp.l)*vp.q1+(vp.kphi1*vp.kphi2/vp.kphi)*((vp.m*vp.g*vp.a1/vp.l)*vp.q2/vp.kphi2p-(vp.m*vp.g*vp.a2/vp.l)*vp.q1/vp.kphi1p))*(1/vp.t1));

% Trasferimento di carico laterale posteriore [N]
deltaZ2 = (((vp.kphi1/vp.kphi)*(vp.m*vp.g)*(vp.h-vp.qb)+(vp.m*vp.g*vp.a1/vp.l)*vp.q1+(vp.kphi1*vp.kphi2/vp.kphi)*((vp.m*vp.g*vp.a2/vp.l)*vp.q2/vp.kphi2p-(vp.m*vp.g*vp.a1/vp.l)*vp.q1/vp.kphi1p))*(1/vp.t1));

% 2) Definizione dei limiti sulle variabili ausiliarie

deltaZ_lim = 1/deltaZ*[-2*vp.m*vp.g 2*vp.m*vp.g];
deltaZ1_lim = 1/deltaZ1*[-2*vp.m*vp.g 2*vp.m*vp.g];
deltaZ2_lim = 1/deltaZ2*[-2*vp.m*vp.g 2*vp.m*vp.g];

% 3) Raggruppamento

% Vettore delle variabili ausiliarie 
Zaus = [deltaZ;deltaZ1;deltaZ2];
% Limiti
Zaus_lim = [deltaZ_lim;deltaZ1_lim;deltaZ2_lim];
Zaus_min = Zaus_lim(:,1);
Zaus_max = Zaus_lim(:,2);

% EQUAZIONI 

% 1) Legge di sterzo

delta11 = -vp.delta10+vp.tau1*deltav+vp.eps1*(vp.t1/(2*vp.l))*(vp.t1*deltav)^2;
delta12 = vp.delta10+vp.tau1*deltav-vp.eps1*(vp.t1/(2*vp.l))*(vp.t1*deltav)^2;
delta21 = -vp.delta20+vp.tau2*deltav+vp.eps2*(vp.t2/(2*vp.l))*(vp.t2*deltav)^2;
delta22 = vp.delta20+vp.tau2*deltav-vp.eps2*(vp.t2/(2*vp.l))*(vp.t2*deltav)^2;

% 2) Velocità pneumatici sistema "Body

% FRONT LEFT
Vb11x = u-(r*vp.t1)/2; Vb11y = v+r*vp.a1;
% FRONT RIGHT
Vb12x = u+(r*vp.t1)/2; Vb12y = v+r*vp.a1;
% REAR LEFT
Vb21x = u-(r*vp.t2)/2; Vb21y = v-r*vp.a2;
% REAR RIGHT
Vb22x = u+(r*vp.t2)/2; Vb22y = v-r*vp.a2;

% 3) Angoli di assetto

% FRONT LEFT
beta11 = (v+r*vp.a1)/(u-r*vp.t1/2);
% FRONT RIGHT
beta12 = (v+r*vp.a1)/(u+r*vp.t1/2);
% REAR LEFT
beta21 = (v-r*vp.a2)/(u-r*vp.t2/2);
% REAR RIGHT
beta22 = (v-r*vp.a2)/(u+r*vp.t2/2);

% 3b) Velocità sistema "Wheel"

% FRONT LEFT
Vw11x = [cos(delta11) sin(delta11)]*[Vb11x;Vb11y];
Vw11y = [-sin(delta11) cos(delta11)]*[Vb11x;Vb11y];
% FRONT RIGHT
Vw12x = [cos(delta12) sin(delta12)]*[Vb12x;Vb12y];
Vw12y = [-sin(delta12) cos(delta12)]*[Vb12x;Vb12y];
% REAR LEFT
Vw21x = [cos(delta21) sin(delta21)]*[Vb21x;Vb21y];
Vw21y = [-sin(delta21) cos(delta21)]*[Vb21x;Vb21y];
% REAR RIGHT
Vw22x = [cos(delta22) sin(delta22)]*[Vb22x;Vb22y];
Vw22y = [-sin(delta22) cos(delta22)]*[Vb22x;Vb22y];

% 4) Angoli di deriva

% FRONT LEFT
alpha11 = delta11-beta11;
% FRONT RIGHT
alpha12 = delta12-beta12;
% REAR LEFT
alpha21 = delta21-beta21;
% REAR RIGHT
alpha22 = delta22-beta22;

% 5) Scorrimenti teorici

% Longitudinali
sigmax11 = (((u-r*vp.t1/2)*cos(delta11)+(v+r*vp.a1)*sin(delta11))-omega11*vp.Rr)/(omega11*vp.Rr);
sigmax12 = (((u+r*vp.t1/2)*cos(delta12)+(v+r*vp.a1)*sin(delta12))-omega12*vp.Rr)/(omega12*vp.Rr);
sigmax21 = (((u-r*vp.t2/2)*cos(delta21)+(v-r*vp.a2)*sin(delta21))-omega21*vp.Rr)/(omega21*vp.Rr);
sigmax22 = (((u+r*vp.t2/2)*cos(delta22)+(v-r*vp.a2)*sin(delta22))-omega22*vp.Rr)/(omega22*vp.Rr);
% Laterali
sigmay11 = ((v+r*vp.a1)*cos(delta11)-(u-r*vp.t1/2)*sin(delta11))/(omega11*vp.Rr);
sigmay12 = ((v+r*vp.a1)*cos(delta12)-(u+r*vp.t1/2)*sin(delta12))/(omega12*vp.Rr);
sigmay21 = ((v-r*vp.a2)*cos(delta21)-(u-r*vp.t2/2)*sin(delta21))/(omega21*vp.Rr);
sigmay22 = ((v-r*vp.a2)*cos(delta22)-(u+r*vp.t2/2)*sin(delta22))/(omega22*vp.Rr);

% 6) Scorrimenti pratici

% SR = slip ratio (quelli lungo x)
% SA = slip angle (quelli lungo y)
SR11 = -(sigmax11/(1+sigmax11));
SR12 = -(sigmax12/(1+sigmax12));
SR21 = -(sigmax21/(1+sigmax21));
SR22 = -(sigmax22/(1+sigmax22));
SA11 = -(sigmay11/(1+sigmax11));
SA12 = -(sigmay12/(1+sigmax12));
SA21 = -(sigmay21/(1+sigmax21));
SA22 = -(sigmay22/(1+sigmax22));

% 7) Aerodinamica

% Resistenza aerodinamica [N]
Xa = 0.5*vp.rho*vp.S*vp.Cx*u^2;

% Deportanza anteriore e posteriore [N]
Z1a = 0.5*vp.rho*vp.S*vp.Cz1*u^2;
Z2a = 0.5*vp.rho*vp.S*vp.Cz2*u^2;

% 8) Carichi sulle ruote

Z10 = vp.m*vp.g*vp.a2/vp.l;
Z20 = vp.m*vp.g*vp.a1/vp.l;

Fz11 = 0.5*(Z10+Z1a-deltaZ)-deltaZ1;
Fz12 = 0.5*(Z10+Z1a-deltaZ)+deltaZ1;
Fz21 = 0.5*(Z20+Z2a+deltaZ)-deltaZ2;
Fz22 = 0.5*(Z20+Z2a+deltaZ)+deltaZ2;

Dx11 = 2.05 * Fz11 - 1.9e-5 * Fz11^2;  % Picco Longitudinale
Dy11 = 1.86 * Fz11 - 2.6e-4 * Fz11^2;  % Picco Laterale
Dx12 = 2.05 * Fz12 - 1.9e-5 * Fz12^2;
Dy12 = 1.86 * Fz12 - 2.6e-4 * Fz12^2;
Dx21 = 2.05 * Fz21 - 1.9e-5 * Fz21^2;
Dy21 = 1.86 * Fz21 - 2.6e-4 * Fz21^2;
Dx22 = 2.05 * Fz22 - 1.9e-5 * Fz22^2;
Dy22 = 1.86 * Fz22 - 2.6e-4 * Fz22^2;

% --- 2. FORZE PURE (Magic Formula base) ---
% Fx0 (Longitudinale)
Bx=45.34; Cx=1.14; Ex=0.55;
Fx011 = Dx11 * sin(Cx * atan(Bx*SR11 - Ex*(Bx*SR11 - atan(Bx*SR11))));
Fx012 = Dx12 * sin(Cx * atan(Bx*SR12 - Ex*(Bx*SR12- atan(Bx*SR12))));
Fx021 = Dx21 * sin(Cx * atan(Bx*SR21 - Ex*(Bx*SR21 - atan(Bx*SR21))));
Fx022 = Dx22 * sin(Cx * atan(Bx*SR22 - Ex*(Bx*SR22 - atan(Bx*SR22))));
% Fy0 (Laterale)
By=20.74; Cy=1.20; Ey=0.48;
Fy011 = Dy11 * sin(Cy * atan(By*SA11 - Ey*(By*SA11 - atan(By*SA11))));
Fy012 = Dy12 * sin(Cy * atan(By*SA12 - Ey*(By*SA12 - atan(By*SA12))));
Fy021 = Dy21 * sin(Cy * atan(By*SA21 - Ey*(By*SA21 - atan(By*SA21))));
Fy022 = Dy22 * sin(Cy * atan(By*SA22 - Ey*(By*SA22 - atan(By*SA22))));
% --- 3. COMBINATO (Ovale di Attrito) ---
% Evita che il vettore forza superi il grip fisico disponibile
Rho = sqrt((Fx011/Dx11)^2 + (Fy011/Dy11)^2);
if Rho > 1
    Scale = 1/Rho;
    Fx11 = Fx011 * Scale;
    Fy11 = Fy011 * Scale;
else
    Fx11 = Fx011;
    Fy11 = Fy011;
end
Rho = sqrt((Fx012/Dx12)^2 + (Fy012/Dy12)^2);
if Rho > 1
    Scale = 1/Rho;
    Fx12 = Fx012 * Scale;
    Fy12 = Fy012 * Scale;
else
    Fx12 = Fx012;
    Fy12 = Fy012;
end
Rho = sqrt((Fx021/Dx21)^2 + (Fy021/Dy21)^2);
if Rho > 1
    Scale = 1/Rho;
    Fx21 = Fx021 * Scale;
    Fy21 = Fy021 * Scale;
else
    Fx21 = Fx021;
    Fy21 = Fy021;
end
Rho = sqrt((Fx022/Dx22)^2 + (Fy022/Dy22)^2);
if Rho > 1
    Scale = 1/Rho;
    Fx22 = Fx022 * Scale;
    Fy22 = Fy022 * Scale;
else
    Fx22 = Fx022;
    Fy22 = Fy022;
end
% --- 4. MOMENTI (Mz, Mx, My) ---
% Mz (Auto-allineamento) - Modellato con MF fittizia
Bmz=8.8; Cmz=2.4; Emz=0.95; Dmz11 = 0.023*Fz11 - 3e-6*Fz11^2;
Dmz12 = 0.023*Fz12 - 3e-6*Fz12^2;
Dmz21 = 0.023*Fz21 - 3e-6*Fz21^2;
Dmz22 = 0.023*Fz22 - 3e-6*Fz22^2;
Mz11_raw = -Dmz11 * sin(Cmz * atan(Bmz*SA11 - Emz*(Bmz*SA11 - atan(Bmz*SA11))));
Mz12_raw = -Dmz12 * sin(Cmz * atan(Bmz*SA12 - Emz*(Bmz*SA12 - atan(Bmz*SA12))));
Mz21_raw = -Dmz21 * sin(Cmz * atan(Bmz*SA21 - Emz*(Bmz*SA21 - atan(Bmz*SA21))));
Mz22_raw = -Dmz22 * sin(Cmz * atan(Bmz*SA22 - Emz*(Bmz*SA22 - atan(Bmz*SA22))));
Mz11 = Mz11_raw*(1-abs(SR11));
Mz12 = Mz12_raw*(1-abs(SR12));
Mz21 = Mz21_raw*(1-abs(SR21));
Mz22 = Mz22_raw*(1-abs(SR22));
% Mx (Ribaltante) - Lineare
Mx11 = -0.024 * Fy11;
Mx12 = -0.024 * Fy12;
Mx21 = -0.024 * Fy21;
Mx22 = -0.024 * Fy22;
% My (Rotolamento) - Costante
My11 = -sign(u) * (0.0024 * Fz11);
My12 = -sign(u) * (0.0024 * Fz12);
My21 = -sign(u) * (0.0024 * Fz21);
My22 = -sign(u) * (0.0024 * Fz22);

% Equazioni di supporto
X11 = Fx11*cos(delta11)-Fy11*sin(delta11);
X12 = Fx12*cos(delta12)-Fy12*sin(delta12);
X21 = Fx21*cos(delta21)-Fy21*sin(delta21);
X22 = Fx22*cos(delta22)-Fy22*sin(delta22);
Y11 = Fx11*sin(delta11)+Fy11*cos(delta11);
Y12 = Fx12*sin(delta12)+Fy12*cos(delta12);
Y21 = Fx21*sin(delta21)+Fy21*cos(delta21);
Y22 = Fx22*sin(delta22)+Fy22*cos(delta22);
X1 = (Fx11*cos(delta11)+Fx12*cos(delta12))-(Fy11*sin(delta11)+Fy12*sin(delta12));
X2 = (Fx21*cos(delta21)+Fx22*cos(delta22))-(Fy21*sin(delta21)+Fy22*sin(delta22));
Y1 = (Fy11*cos(delta11)+Fy12*cos(delta12))+(Fx11*sin(delta11)+Fx12*sin(delta12));
Y2 = (Fy21*cos(delta21)+Fy22*cos(delta22))+(Fx21*sin(delta21)+Fx22*sin(delta22));
deltaX1 = ((Fx12*cos(delta12)-Fx11*cos(delta11))-(Fy12*sin(delta12)-Fy11*sin(delta11)))/2;
deltaX2 = ((Fx22*cos(delta22)-Fx21*cos(delta21))-(Fy22*sin(delta22)-Fy21*sin(delta21)))/2;

% Ruote Anteriori (11 = FL, 12 = FR)
% Nelle Formula SAE a trazione posteriore, qui arriva solo la frenata
T11 = Tbrake / 4; 
T12 = Tbrake / 4;

% Ruote Posteriori (21 = RL, 22 = RR)
% Qui arriva la coppia motrice (Tdrive) divisa dal differenziale + la frenata
T21 = TdriveL + (Tbrake / 4);
T22 = TdriveR + (Tbrake / 4);

% Derivate
dot_u = (((X1+X2-Xa)/vp.m)+v*r);
dot_v = (((Y1+Y2)/vp.m)-u*r);
dot_r = ((Y1*vp.a1-Y2*vp.a2+deltaX1*vp.t1+deltaX2*vp.t2)/vp.Jz);
dot_nu = (u*sin(epsilon)+v*cos(epsilon));
dot_epsilon = r;
dot_omega11 = ((T11-Fx11*vp.Rr)/vp.tyre.IYY);
dot_omega12 = ((T12-Fx12*vp.Rr)/vp.tyre.IYY);
dot_omega21 = ((T21-Fx21*vp.Rr)/vp.tyre.IYY);
dot_omega22 = ((T22-Fx22*vp.Rr)/vp.tyre.IYY);
% Scalatura
dot_x = [dot_u; dot_v; dot_r; dot_nu; dot_epsilon; 
            dot_omega11; dot_omega12; dot_omega21; dot_omega22];

out = dot_x;

end

== matlab function TV_Sim_Track_Copia/MATLAB Function3 ==
  data: T_L output; T_req input; T_R output; Mz_ctrl input; vp parameter
function [T_L, T_R]  = torque_allocator(T_req, Mz_ctrl, vp)

deltaT = (Mz_ctrl * vp.Rr) / vp.t2;

T_R = T_req/2 + deltaT;
T_L = T_req/2 - deltaT;

T_R = min(vp.Tdrivemax, max(-vp.Tregenmax, T_R));
T_L = min(vp.Tdrivemax, max(-vp.Tregenmax, T_L));

== matlab function TV_Sim_Track_Copia/MATLAB Function4 ==
  data: u input; out output; v input; r input; psi input
function out = XY_pos(u, v, r, psi)

X_dot = u*cos(psi) - v*sin(psi);
Y_dot = u*sin(psi) + v*cos(psi);
psi_dot = r;

out = [X_dot, Y_dot, psi_dot];

== matlab function TV_Sim_Track_Copia/MATLAB Function5 ==
  data: u input; out output; v input; r input; psi input
function out = XY_pos(u, v, r, psi)

X_dot = u*cos(psi) - v*sin(psi);
Y_dot = u*sin(psi) + v*cos(psi);
psi_dot = r;

out = [X_dot, Y_dot, psi_dot];
